simulink model "ff_ccc_"  (R2024b)
settings: Solver=FixedStepAuto  StartTime=0.0  StopTime=Ts  FixedStep=Ts  RelTol=1e-3
InitFcn:
  | load('.\data_smk_\ff_c_controller_parameters.mat')
settings Model: Creator=rmrane  LastModifiedBy=vreyesdreke
settings OptimizationCC: DefaultParameterBehavior=Inlined  EnhancedBackFolding=on  PassReuseOutputArgsAs=Individual arguments  ZeroExternalMemoryAtStartup=off  ZeroInternalMemoryAtStartup=off  OptimizeBlockOrder=speed  DifferentSizesBufferReuse=on  OptimizationCustomize=off  EfficientTunableParamExpr=on
settings DebuggingCC: ParameterTunabilityLossMsg=error
settings SFSimCC: MATLABDynamicMemAlloc=off
settings RTWCC: Description=Embedded Coder  SystemTargetFile=ert.tlc  TemplateMakefile=ert_default_tmf
settings CodeAppCC: GenerateComments=off  IgnoreCustomStorageClasses=off  OperatorAnnotations=on  SimulinkDataObjDesc=on  SFDataObjDesc=on  CustomSymbolStrType=$N$R$M  SimulinkBlockComments=off  InternalIdentifier=Classic
settings ERTTargetCC: GenerateSampleERTMain=on  SupportAbsoluteTime=off  SupportNonFinite=off  SupportComplex=off  ERTCustomFileTemplate=example_file_process.tlc  ConvertIfToSwitch=off  SuppressUnreachableDefaultCases=off  EnableSignedLeftShifts=off  EnableSignedRightShifts=off  DynamicArrayContainerType=coder::array

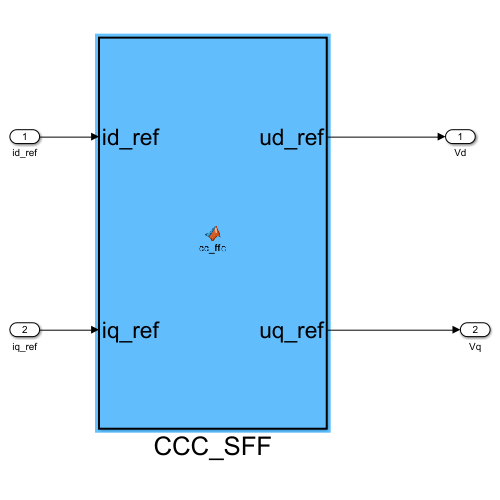
[thumbnail: Simulink's stored preview of the top-level diagram]
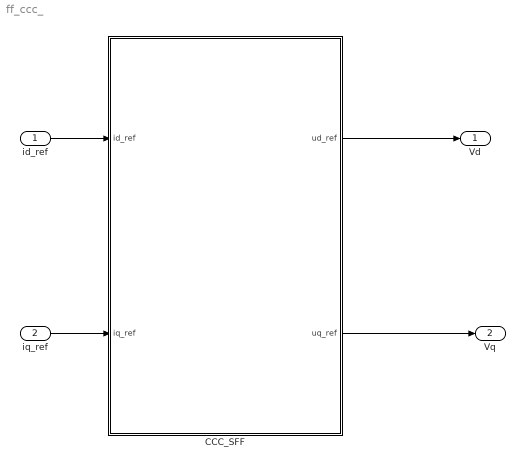
== system ff_ccc_ ==
  id_ref : Inport
  iq_ref : Inport  Port=2
  CCC_SFF : MATLAB Function  TreatAsAtomicUnit=on
  Vd : Outport
  Vq : Outport  Port=2
  wires:
  CCC_SFF/1(ud_ref) -> Vd/1
  CCC_SFF/2(uq_ref) -> Vq/1
  id_ref/1 -> CCC_SFF/1(id_ref)
  iq_ref/1 -> CCC_SFF/2(iq_ref)

== matlab function ff_ccc_/CCC_SFF ==
  settings: updateMethod=DISCRETE  sampleTime=Ts
  data: id_ref input size=1; ud_ref output size=1; uq_ref output size=1; iq_ref input size=1
function [ud_ref,uq_ref] = cc_ffc(id_ref,iq_ref)
    % oc_ffc(id_ref,iq_ref) feedforward controller gain.
    m_ss = coder.load('.\data_smk_\ff_c_controller_parameters.mat','-mat','-regexp','Kff');
    uss = m_ss.Kff*[id_ref,iq_ref]';
    ud_ref = uss(1);
    uq_ref = uss(2);
end
